simulink model "segway_completo"  (R2023b)
settings: Solver=ode45  StartTime=0.0  StopTime=8  MaxStep=1e-3  RelTol=1e-9  AbsTol=1e-11
values from neighbouring files (symbols this model uses):
  acople_rotor = p.e_acople    [INICIAR_SEGWAY.m]
  b_eje_mecanico = p.b_eje_mecanico    [INICIAR_SEGWAY.m]
  b_m_motor = motor.b_m    / motor.n_motores    [INICIAR_SEGWAY.m]
  b_phi = p.b_phi    [INICIAR_SEGWAY.m]
  b_x = p.b_x    [INICIAR_SEGWAY.m]
  beta_V_motor = motor.beta_V / motor.n_motores    [INICIAR_SEGWAY.m]
  compensar_delta_G = 1    [INICIAR_SEGWAY.m]
  giro_ref = 0    [INICIAR_SEGWAY.m]
  K = C.K    [INICIAR_SEGWAY.m]
  Kp_servo = 12    [INICIAR_SEGWAY.m]
  omega0 = 0    [INICIAR_SEGWAY.m]
  phi0 = deg2rad(5)    [INICIAR_SEGWAY.m]
  r = p.r    [INICIAR_SEGWAY.m]
  ruido_encoder_v = 0    [INICIAR_SEGWAY.m]
  ruido_encoder_x = 0    [INICIAR_SEGWAY.m]
  ruido_imu_angulo = 0    [INICIAR_SEGWAY.m]
  ruido_imu_giro = 0    [INICIAR_SEGWAY.m]
  sesgo_imu = 0    [INICIAR_SEGWAY.m]
  t_consigna = 2.0    (= 2)    [INICIAR_SEGWAY.m]
  t_patas = 4.0    (= 4)    [INICIAR_SEGWAY.m]
  tabla_a = zeros(size(tabla_theta))    [INICIAR_SEGWAY.m]
  tabla_delta_G = zeros(size(tabla_theta))    [INICIAR_SEGWAY.m]
  tabla_h = zeros(size(tabla_theta))    [INICIAR_SEGWAY.m]
  tabla_j = zeros(size(tabla_theta))    [INICIAR_SEGWAY.m]
  tabla_k = zeros(size(tabla_theta))    [INICIAR_SEGWAY.m]
  tabla_theta = deg2rad(grados_tabla(:))    [INICIAR_SEGWAY.m]
  tau_traccion = limite_de_traccion(p)    [INICIAR_SEGWAY.m]
  theta_pata_0 = deg2rad(postura_deg)    [INICIAR_SEGWAY.m]
  theta_pata_fin = deg2rad(theta_pata_fin)    [INICIAR_SEGWAY.m]
  theta_pata_max = (360 - min(fisicos.th))*pi/180    [INICIAR_SEGWAY.m]
  theta_pata_min = (360 - max(fisicos.th))*pi/180    [INICIAR_SEGWAY.m]
  Ts_sensores = 0.005    [INICIAR_SEGWAY.m]
  v0 = 0    [INICIAR_SEGWAY.m]
  V_bat = motor.V_bat    [INICIAR_SEGWAY.m]
  w_servo_max = deg2rad(300)    [INICIAR_SEGWAY.m]
  x0 = 0    [INICIAR_SEGWAY.m]
  x_destino = 0.30    (= 0.3)    [INICIAR_SEGWAY.m]
libraries: simulink x2
settings Model: Creator=calde  LastModifiedBy=calde

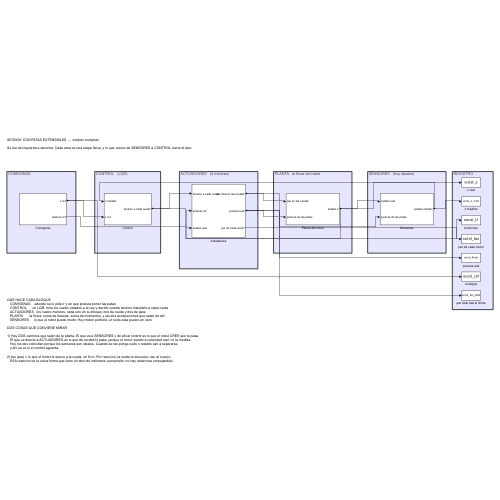
[thumbnail: Simulink's stored preview of the top-level diagram]
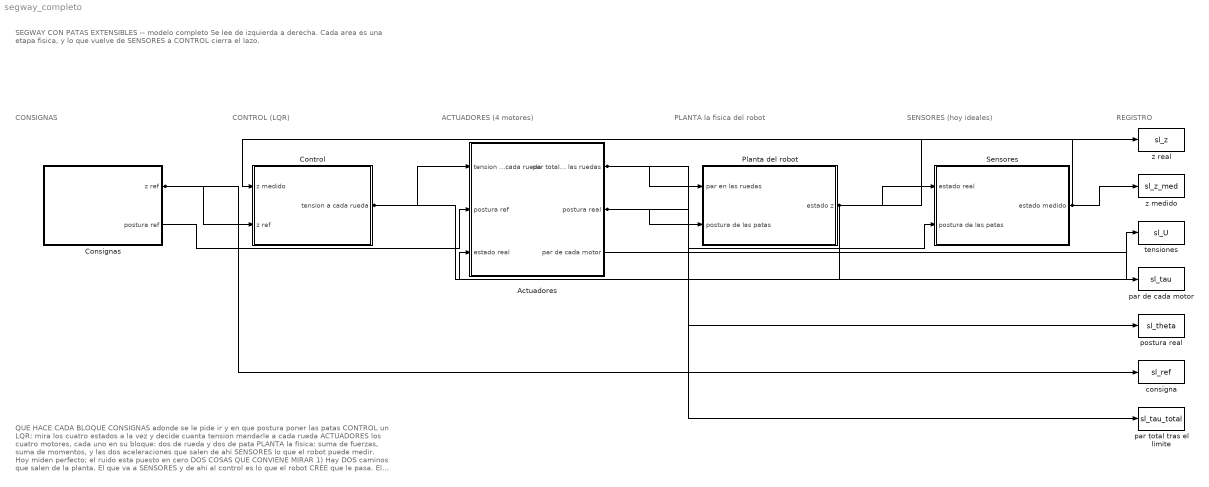
== system segway_completo ==
  note: CONSIGNAS
  note: CONTROL (LQR)
  note: ACTUADORES (4 motores)
  note: PLANTA la fisica del robot
  note: SENSORES (hoy ideales)
  note: REGISTRO
  note: SEGWAY CON PATAS EXTENSIBLES  --  modelo completo
      |
      | Se lee de izquierda a derecha. Cada area es una etapa fisica, y lo que vuelve de SENSORES a CONTROL cierra el lazo.
  note: QUE HACE CADA BLOQUE
      |    CONSIGNAS    adonde se le pide ir y en que postura poner las patas
      |    CONTROL      un LQR: mira los cuatro estados a la vez y decide cuanta tension mandarle a cada rueda
      |    ACTUADORES   los cuatro motores, cada uno en su bloque: dos de rueda y dos de pata
      |    PLANTA       la fisica: suma de fuerzas, suma de momentos, y las dos aceleraciones que salen de ahi
      |    SENSORES     lo que el robot puede medir. Hoy miden perfecto; el ruido esta puesto en cero
      |
      | DOS COSAS QUE CONVIENE MIRAR
      |
      | 1) Hay DOS caminos que salen de la planta. El que va a SENSORES y de ahi al control es lo que el robot CREE que le pasa.
      |    El que va directo a ACTUADORES es lo que de verdad le pasa, porque el motor siente la velocidad real, no la medida.
      |    Hoy los dos coinciden porque los sensores son ideales. Cuando se les ponga ruido o retardo van a separarse,
      |    y ahi se ve si el control aguanta.
      |
      | 2) tau (par) = lo que el motor le tuerce a la rueda, en N m. Por reaccion, la rueda le devuelve -tau al cuerpo.
      |    ESA reaccion es la unica forma que tiene el robot de inclinarse a proposito: no hay nada mas empujandolo.
  Actuadores : Subsystem
  Consignas : Subsystem
  Control : Subsystem
  Planta del robot : Subsystem
  Sensores : Subsystem
  consigna : ToWorkspace  VariableName=sl_ref  SaveFormat=Structure With Time  SampleTime=-1
  par de cada motor : ToWorkspace  VariableName=sl_tau  SaveFormat=Structure With Time  SampleTime=-1
  par total tras el limite : ToWorkspace  VariableName=sl_tau_total  SaveFormat=Structure With Time  SampleTime=-1
  postura real : ToWorkspace  VariableName=sl_theta  SaveFormat=Structure With Time  SampleTime=-1
  tensiones : ToWorkspace  VariableName=sl_U  SaveFormat=Structure With Time  SampleTime=-1
  z medido : ToWorkspace  VariableName=sl_z_med  SaveFormat=Structure With Time  SampleTime=-1
  z real : ToWorkspace  VariableName=sl_z  SaveFormat=Structure With Time  SampleTime=-1
  wires:
  Consignas/1(z ref) -> Control/2(z ref), consigna/1
  Consignas/2(postura ref) -> Actuadores/2(postura ref)
  Sensores/1(estado medido) -> Control/1(z medido), z medido/1
  Control/1(tension a cada rueda) -> Actuadores/1(tension a cada rueda), tensiones/1
  Planta del robot/1(estado z) -> Actuadores/3(estado real), Sensores/1(estado real), z real/1
  Actuadores/1(par total en las ruedas) -> Planta del robot/1(par en las ruedas), par total tras el limite/1
  Actuadores/2(postura real) -> Planta del robot/2(postura de las patas), Sensores/2(postura de las patas), postura real/1
  Actuadores/3(par de cada motor) -> par de cada motor/1

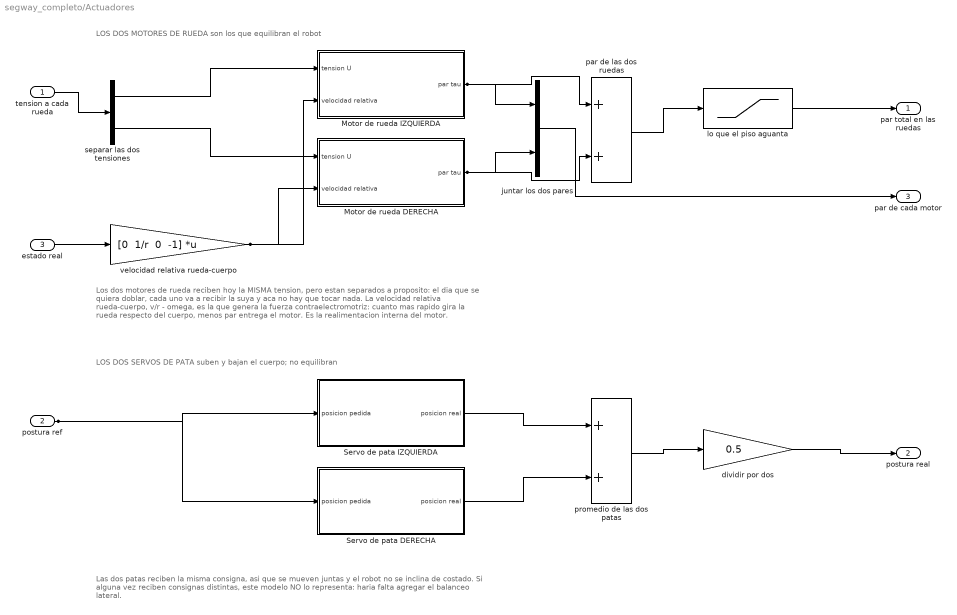
== system segway_completo/Actuadores ==
  note: LOS DOS MOTORES DE RUEDA son los que equilibran el robot
  note: LOS DOS SERVOS DE PATA suben y bajan el cuerpo; no equilibran
  note: Los dos motores de rueda reciben hoy la MISMA tension, pero estan separados a proposito: el dia que se
      | quiera doblar, cada uno va a recibir la suya y aca no hay que tocar nada.
      |
      | La velocidad relativa rueda-cuerpo, v/r - omega, es la que genera la fuerza contraelectromotriz: cuanto mas
      | rapido gira la rueda respecto del cuerpo, menos par entrega el motor. Es la realimentacion interna del motor.
  note: Las dos patas reciben la misma consigna, asi que se mueven juntas y el robot no se inclina de costado.
      | Si alguna vez reciben consignas distintas, este modelo NO lo representa: haria falta agregar el balanceo lateral.
  tension a cada rueda : Inport
  postura ref : Inport  Port=2
  estado real : Inport  Port=3
  Motor de rueda DERECHA : Subsystem
  Motor de rueda IZQUIERDA : Subsystem
  Servo de pata DERECHA : Subsystem
  Servo de pata IZQUIERDA : Subsystem
  dividir por dos : Gain  Gain=0.5
  juntar los dos pares : Mux  Inputs=2
  lo que el piso aguanta : Saturate  UpperLimit=tau_traccion  LowerLimit=-tau_traccion
  par de las dos ruedas : Sum
  promedio de las dos patas : Sum
  separar las dos tensiones : Demux  Outputs=2
  velocidad relativa rueda-cuerpo : Gain  Gain="[0  1/r  0  -1]"  Multiplication=Matrix(K*u)
  par total en las ruedas : Outport
  postura real : Outport  Port=2
  par de cada motor : Outport  Port=3
  wires:
  tension a cada rueda/1 -> separar las dos tensiones/1
  estado real/1 -> velocidad relativa rueda-cuerpo/1
  separar las dos tensiones/1 -> Motor de rueda IZQUIERDA/1(tension U)
  separar las dos tensiones/2 -> Motor de rueda DERECHA/1(tension U)
  velocidad relativa rueda-cuerpo/1 -> Motor de rueda IZQUIERDA/2(velocidad relativa), Motor de rueda DERECHA/2(velocidad relativa)
  Motor de rueda IZQUIERDA/1(par tau) -> par de las dos ruedas/1, juntar los dos pares/1
  Motor de rueda DERECHA/1(par tau) -> par de las dos ruedas/2, juntar los dos pares/2
  juntar los dos pares/1 -> par de cada motor/1
  par de las dos ruedas/1 -> lo que el piso aguanta/1
  lo que el piso aguanta/1 -> par total en las ruedas/1
  postura ref/1 -> Servo de pata IZQUIERDA/1(posicion pedida), Servo de pata DERECHA/1(posicion pedida)
  Servo de pata IZQUIERDA/1(posicion real) -> promedio de las dos patas/1
  Servo de pata DERECHA/1(posicion real) -> promedio de las dos patas/2
  promedio de las dos patas/1 -> dividir por dos/1
  dividir por dos/1 -> postura real/1

== system segway_completo/Consignas ==
  note: EQUILIBRIO Y POSICION: z_ref = [x deseado ; 0 ; 0 ; 0]
  note: PATAS: angulo pedido al servo, en radianes (10 grados = plegada, 40 = estirada)
  note: Por defecto la postura es constante, asi que el robot se comporta como el modelo verificado.
      | Si se le pone un escalon (theta_pata_fin distinto de theta_pata_0) las patas se mueven y
      | cambian la altura del cuerpo: ver el capitulo 9 del PDF del modelo.
  adonde ir : Step  Time=t_consigna  After=x_destino  SampleTime=0
  armar z ref : Mux  Inputs=2
  postura de las patas : Step  Time=t_patas  Before=theta_pata_0  After=theta_pata_fin  SampleTime=0
  "velocidad, angulo y giro pedidos" : Constant  Value=[0; 0; 0]
  z ref : Outport
  postura ref : Outport  Port=2
  wires:
  adonde ir/1 -> armar z ref/1
  "velocidad, angulo y giro pedidos"/1 -> armar z ref/2
  armar z ref/1 -> z ref/1
  postura de las patas/1 -> postura ref/1

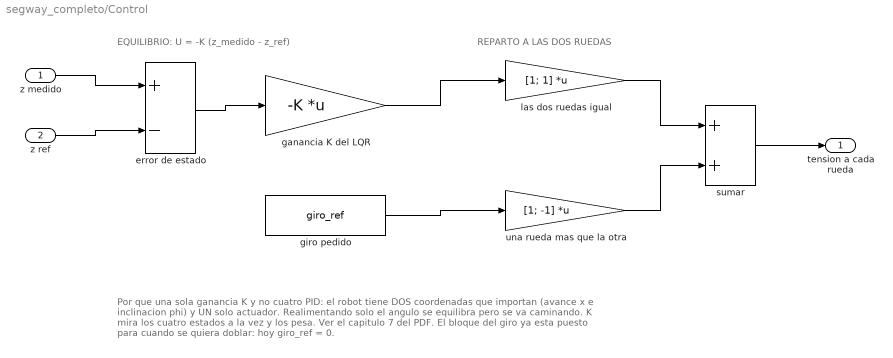
== system segway_completo/Control ==
  note: EQUILIBRIO: U = -K (z_medido - z_ref)
  note: REPARTO A LAS DOS RUEDAS
  note: Por que una sola ganancia K y no cuatro PID: el robot tiene DOS coordenadas que importan
      | (avance x e inclinacion phi) y UN solo actuador. Realimentando solo el angulo se equilibra
      | pero se va caminando. K mira los cuatro estados a la vez y los pesa. Ver el capitulo 7 del PDF.
      |
      | El bloque del giro ya esta puesto para cuando se quiera doblar: hoy giro_ref = 0.
  z medido : Inport
  z ref : Inport  Port=2
  error de estado : Sum  Inputs=+-
  ganancia K del LQR : Gain  Gain=-K  Multiplication=Matrix(K*u)
  giro pedido : Constant  Value=giro_ref
  las dos ruedas igual : Gain  Gain=[1; 1]  Multiplication=Matrix(K*u)
  sumar : Sum
  una rueda mas que la otra : Gain  Gain=[1; -1]  Multiplication=Matrix(K*u)
  tension a cada rueda : Outport
  wires:
  z medido/1 -> error de estado/1
  z ref/1 -> error de estado/2
  error de estado/1 -> ganancia K del LQR/1
  ganancia K del LQR/1 -> las dos ruedas igual/1
  giro pedido/1 -> una rueda mas que la otra/1
  las dos ruedas igual/1 -> sumar/1
  una rueda mas que la otra/1 -> sumar/2
  sumar/1 -> tension a cada rueda/1

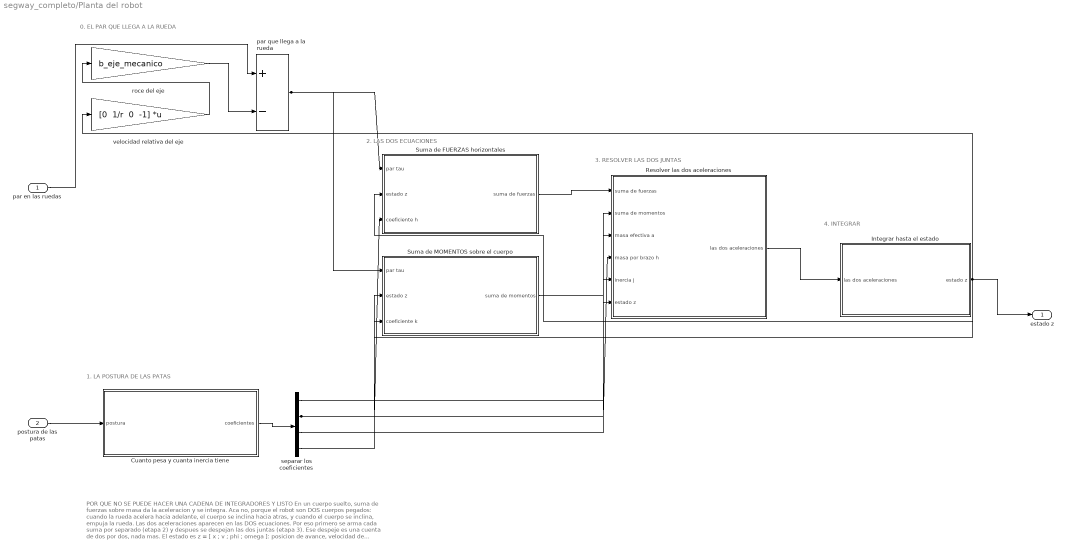
== system segway_completo/Planta del robot ==
  note: 1. LA POSTURA DE LAS PATAS
  note: 0. EL PAR QUE LLEGA A LA RUEDA
  note: 2. LAS DOS ECUACIONES
  note: 3. RESOLVER LAS DOS JUNTAS
  note: 4. INTEGRAR
  note: POR QUE NO SE PUEDE HACER UNA CADENA DE INTEGRADORES Y LISTO
      |
      | En un cuerpo suelto, suma de fuerzas sobre masa da la aceleracion y se integra. Aca no, porque el robot son DOS cuerpos
      | pegados: cuando la rueda acelera hacia adelante, el cuerpo se inclina hacia atras, y cuando el cuerpo se inclina, empuja
      | la rueda. Las dos aceleraciones aparecen en las DOS ecuaciones. Por eso primero se arma cada suma por separado (etapa 2)
      | y despues se despejan las dos juntas (etapa 3). Ese despeje es una cuenta de dos por dos, nada mas.
      |
      | El estado es  z = [ x ; v ; phi ; omega ]:  posicion de avance, velocidad de avance, inclinacion y velocidad de inclinacion.
  par en las ruedas : Inport
  postura de las patas : Inport  Port=2
  Cuanto pesa y cuanta inercia tiene : Subsystem
  Integrar hasta el estado : Subsystem
  Resolver las dos aceleraciones : Subsystem
  Suma de FUERZAS horizontales : Subsystem
  Suma de MOMENTOS sobre el cuerpo : Subsystem
  par que llega a la rueda : Sum  Inputs=+-
  roce del eje : Gain  Gain=b_eje_mecanico
  separar los coeficientes : Demux
  velocidad relativa del eje : Gain  Gain="[0  1/r  0  -1]"  Multiplication=Matrix(K*u)
  estado z : Outport
  wires:
  postura de las patas/1 -> Cuanto pesa y cuanta inercia tiene/1(postura)
  Cuanto pesa y cuanta inercia tiene/1(coeficientes) -> separar los coeficientes/1
  Integrar hasta el estado/1(estado z) -> velocidad relativa del eje/1, Suma de FUERZAS horizontales/2(estado z), Suma de MOMENTOS sobre el cuerpo/2(estado z), Resolver las dos aceleraciones/6(estado z), estado z/1
  velocidad relativa del eje/1 -> roce del eje/1
  par en las ruedas/1 -> par que llega a la rueda/1
  roce del eje/1 -> par que llega a la rueda/2
  par que llega a la rueda/1 -> Suma de FUERZAS horizontales/1(par tau), Suma de MOMENTOS sobre el cuerpo/1(par tau)
  separar los coeficientes/2 -> Suma de FUERZAS horizontales/3(coeficiente h), Resolver las dos aceleraciones/4(masa por brazo h)
  separar los coeficientes/4 -> Suma de MOMENTOS sobre el cuerpo/3(coeficiente k)
  Suma de FUERZAS horizontales/1(suma de fuerzas) -> Resolver las dos aceleraciones/1(suma de fuerzas)
  Suma de MOMENTOS sobre el cuerpo/1(suma de momentos) -> Resolver las dos aceleraciones/2(suma de momentos)
  separar los coeficientes/1 -> Resolver las dos aceleraciones/3(masa efectiva a)
  separar los coeficientes/3 -> Resolver las dos aceleraciones/5(inercia j)
  Resolver las dos aceleraciones/1(las dos aceleraciones) -> Integrar hasta el estado/1(las dos aceleraciones)

== system segway_completo/Sensores ==
  note: ENCODERS: x y v
  note: IMU: phi y omega
  note: HOY LOS SENSORES SON IDEALES: miden exactamente lo que pasa y el ruido esta en cero. Por eso la senal que
      | entra al control es identica a la real, y el resultado coincide con el modelo matematico.
      |
      | Los lugares donde meter la realidad ya estan puestos:
      |   - ruido: las variables ruido_* valen cero; poniendoles un numero aparece el ruido de medicion
      |   - sesgo de la IMU: sesgo_imu, en radianes
      |   - compensacion de la postura: compensar_delta_G vale 1; poniendolo en 0 se ve el error de no corregirla
      |
      | Lo que TODAVIA no esta y hay que agregar antes de pasar a firmware: periodo de muestreo, retardo de calculo
      | y cuantizacion del encoder. Con esos tres el LQR hubo que repesarlo (capitulo 7 del PDF).
  estado real : Inport
  postura de las patas : Inport  Port=2
  Encoders de las ruedas : Subsystem
  IMU MPU-6050 : Subsystem
  armar el estado medido : Mux  Inputs=2
  estado medido : Outport
  wires:
  estado real/1 -> Encoders de las ruedas/1(estado real), IMU MPU-6050/1(estado real)
  postura de las patas/1 -> IMU MPU-6050/2(postura de las patas)
  Encoders de las ruedas/1(x y v medidos) -> armar el estado medido/1
  IMU MPU-6050/1(phi y omega medidos) -> armar el estado medido/2
  armar el estado medido/1 -> estado medido/1

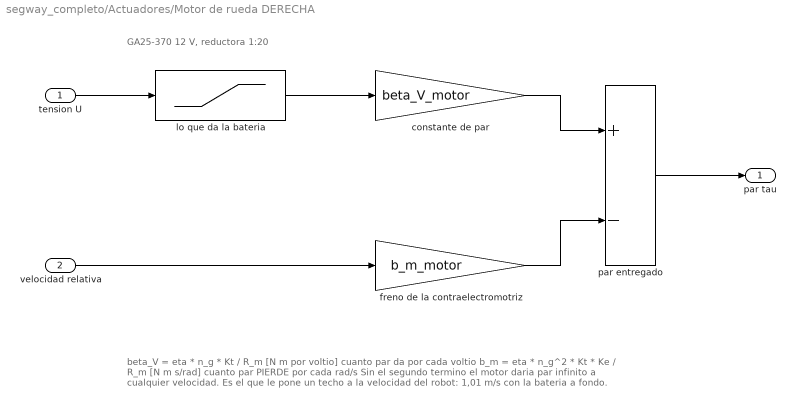
== system segway_completo/Actuadores/Motor de rueda DERECHA ==
  note: GA25-370 12 V, reductora 1:20
  note: beta_V = eta * n_g * Kt / R_m   [N m por voltio]        cuanto par da por cada voltio
      | b_m    = eta * n_g^2 * Kt * Ke / R_m   [N m s/rad]      cuanto par PIERDE por cada rad/s
      |
      | Sin el segundo termino el motor daria par infinito a cualquier velocidad. Es el que le pone
      | un techo a la velocidad del robot: 1,01 m/s con la bateria a fondo.
  tension U : Inport
  velocidad relativa : Inport  Port=2
  constante de par : Gain  Gain=beta_V_motor
  freno de la contraelectromotriz : Gain  Gain=b_m_motor
  lo que da la bateria : Saturate  UpperLimit=V_bat  LowerLimit=-V_bat
  par entregado : Sum  Inputs=+-
  par tau : Outport
  wires:
  tension U/1 -> lo que da la bateria/1
  lo que da la bateria/1 -> constante de par/1
  velocidad relativa/1 -> freno de la contraelectromotriz/1
  constante de par/1 -> par entregado/1
  freno de la contraelectromotriz/1 -> par entregado/2
  par entregado/1 -> par tau/1

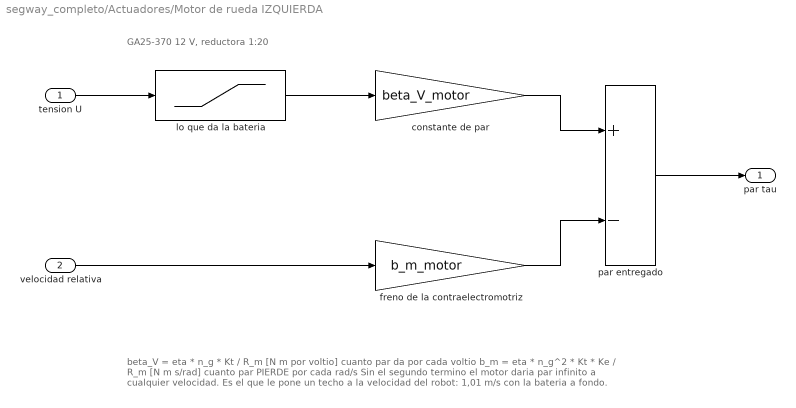
== system segway_completo/Actuadores/Motor de rueda IZQUIERDA ==
  note: GA25-370 12 V, reductora 1:20
  note: beta_V = eta * n_g * Kt / R_m   [N m por voltio]        cuanto par da por cada voltio
      | b_m    = eta * n_g^2 * Kt * Ke / R_m   [N m s/rad]      cuanto par PIERDE por cada rad/s
      |
      | Sin el segundo termino el motor daria par infinito a cualquier velocidad. Es el que le pone
      | un techo a la velocidad del robot: 1,01 m/s con la bateria a fondo.
  tension U : Inport
  velocidad relativa : Inport  Port=2
  constante de par : Gain  Gain=beta_V_motor
  freno de la contraelectromotriz : Gain  Gain=b_m_motor
  lo que da la bateria : Saturate  UpperLimit=V_bat  LowerLimit=-V_bat
  par entregado : Sum  Inputs=+-
  par tau : Outport
  wires:
  tension U/1 -> lo que da la bateria/1
  lo que da la bateria/1 -> constante de par/1
  velocidad relativa/1 -> freno de la contraelectromotriz/1
  constante de par/1 -> par entregado/1
  freno de la contraelectromotriz/1 -> par entregado/2
  par entregado/1 -> par tau/1

== system segway_completo/Actuadores/Servo de pata DERECHA ==
  note: DS3240 40 kg cm: lazo de posicion
  note: Un servo de posicion ya trae su propio control adentro: por eso aca no hay que disenarle nada,
      | solo decirle a que angulo ir. El lazo que se ve es el que el servo tiene de fabrica.
      |
      | Los topes del integrador son los topes MECANICOS de la pata: 10 grados plegada, 40 estirada.
      | Que esten en el integrador y no en una saturacion aparte evita que el angulo se pase y despues vuelva.
  posicion pedida : Inport
  angulo de la pata : Integrator  InitialCondition=theta_pata_0  LimitOutput=on  UpperSaturationLimit=theta_pata_max  LowerSaturationLimit=theta_pata_min
  error de posicion : Sum  Inputs=+-
  ganancia del servo : Gain  Gain=Kp_servo
  velocidad maxima : Saturate  UpperLimit=w_servo_max  LowerLimit=-w_servo_max
  posicion real : Outport
  wires:
  posicion pedida/1 -> error de posicion/1
  ganancia del servo/1 -> velocidad maxima/1
  error de posicion/1 -> ganancia del servo/1
  velocidad maxima/1 -> angulo de la pata/1
  angulo de la pata/1 -> posicion real/1, error de posicion/2

== system segway_completo/Actuadores/Servo de pata IZQUIERDA ==
  note: DS3240 40 kg cm: lazo de posicion
  note: Un servo de posicion ya trae su propio control adentro: por eso aca no hay que disenarle nada,
      | solo decirle a que angulo ir. El lazo que se ve es el que el servo tiene de fabrica.
      |
      | Los topes del integrador son los topes MECANICOS de la pata: 10 grados plegada, 40 estirada.
      | Que esten en el integrador y no en una saturacion aparte evita que el angulo se pase y despues vuelva.
  posicion pedida : Inport
  angulo de la pata : Integrator  InitialCondition=theta_pata_0  LimitOutput=on  UpperSaturationLimit=theta_pata_max  LowerSaturationLimit=theta_pata_min
  error de posicion : Sum  Inputs=+-
  ganancia del servo : Gain  Gain=Kp_servo
  velocidad maxima : Saturate  UpperLimit=w_servo_max  LowerLimit=-w_servo_max
  posicion real : Outport
  wires:
  posicion pedida/1 -> error de posicion/1
  ganancia del servo/1 -> velocidad maxima/1
  error de posicion/1 -> ganancia del servo/1
  velocidad maxima/1 -> angulo de la pata/1
  angulo de la pata/1 -> posicion real/1, error de posicion/2

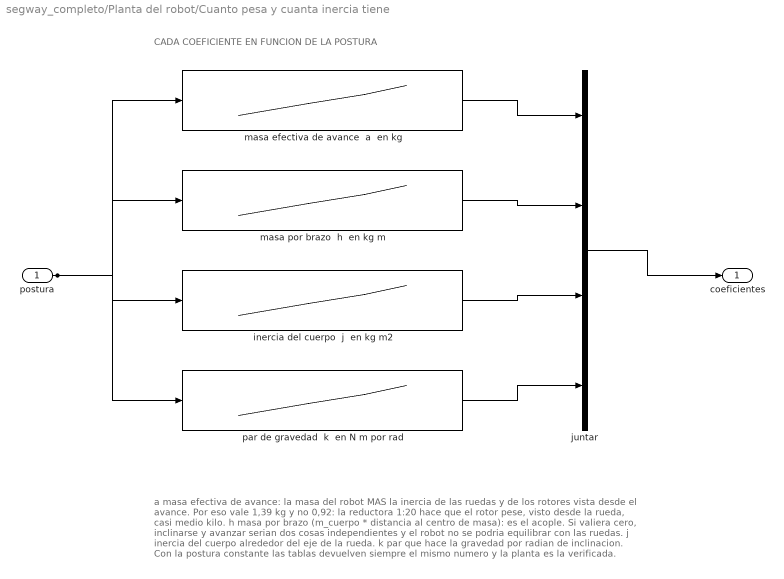
== system segway_completo/Planta del robot/Cuanto pesa y cuanta inercia tiene ==
  note: CADA COEFICIENTE EN FUNCION DE LA POSTURA
  note: a  masa efectiva de avance: la masa del robot MAS la inercia de las ruedas y de los rotores vista desde el avance.
      |    Por eso vale 1,39 kg y no 0,92: la reductora 1:20 hace que el rotor pese, visto desde la rueda, casi medio kilo.
      |
      | h  masa por brazo (m_cuerpo * distancia al centro de masa): es el acople. Si valiera cero, inclinarse y avanzar
      |    serian dos cosas independientes y el robot no se podria equilibrar con las ruedas.
      |
      | j  inercia del cuerpo alrededor del eje de la rueda.      k  par que hace la gravedad por radian de inclinacion.
      |
      | Con la postura constante las tablas devuelven siempre el mismo numero y la planta es la verificada.
  postura : Inport
  inercia del cuerpo  j  en kg m2 : Lookup_n-D  NumberOfTableDimensions=1  BreakpointsForDimension1=tabla_theta  Table=tabla_j  InternalRulePriority=Speed  RndMeth=Simplest
  juntar : Mux
  masa efectiva de avance  a  en kg : Lookup_n-D  NumberOfTableDimensions=1  BreakpointsForDimension1=tabla_theta  Table=tabla_a  InternalRulePriority=Speed  RndMeth=Simplest
  masa por brazo  h  en kg m : Lookup_n-D  NumberOfTableDimensions=1  BreakpointsForDimension1=tabla_theta  Table=tabla_h  InternalRulePriority=Speed  RndMeth=Simplest
  par de gravedad  k  en N m por rad : Lookup_n-D  NumberOfTableDimensions=1  BreakpointsForDimension1=tabla_theta  Table=tabla_k  InternalRulePriority=Speed  RndMeth=Simplest
  coeficientes : Outport
  wires:
  postura/1 -> masa efectiva de avance  a  en kg/1, masa por brazo  h  en kg m/1, inercia del cuerpo  j  en kg m2/1, par de gravedad  k  en N m por rad/1
  masa efectiva de avance  a  en kg/1 -> juntar/1
  masa por brazo  h  en kg m/1 -> juntar/2
  inercia del cuerpo  j  en kg m2/1 -> juntar/3
  par de gravedad  k  en N m por rad/1 -> juntar/4
  juntar/1 -> coeficientes/1

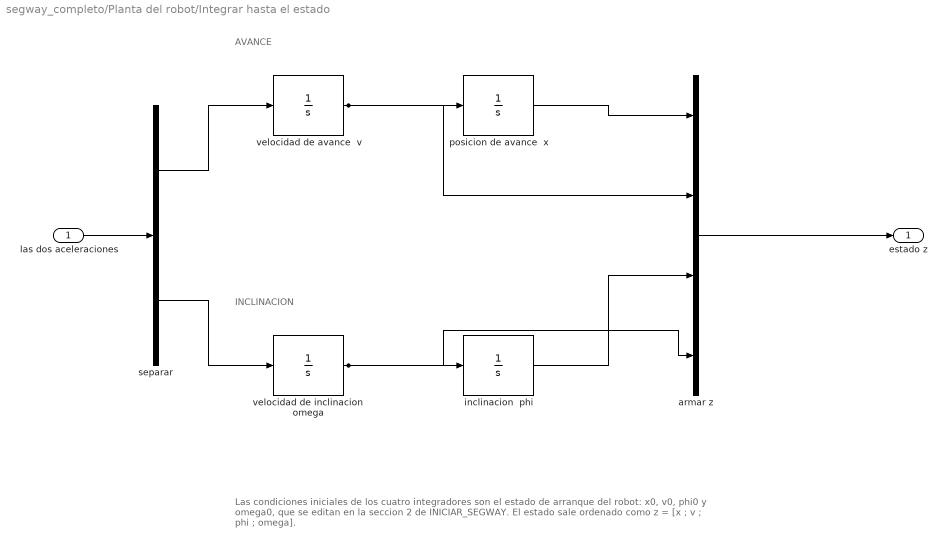
== system segway_completo/Planta del robot/Integrar hasta el estado ==
  note: AVANCE
  note: INCLINACION
  note: Las condiciones iniciales de los cuatro integradores son el estado de arranque del robot:
      | x0, v0, phi0 y omega0, que se editan en la seccion 2 de INICIAR_SEGWAY.
      | El estado sale ordenado como z = [x ; v ; phi ; omega].
  las dos aceleraciones : Inport
  armar z : Mux
  inclinacion  phi : Integrator  InitialCondition=phi0
  posicion de avance  x : Integrator  InitialCondition=x0
  separar : Demux  Outputs=2
  velocidad de avance  v : Integrator  InitialCondition=v0
  velocidad de inclinacion  omega : Integrator  InitialCondition=omega0
  estado z : Outport
  wires:
  las dos aceleraciones/1 -> separar/1
  separar/1 -> velocidad de avance  v/1
  velocidad de avance  v/1 -> posicion de avance  x/1, armar z/2
  separar/2 -> velocidad de inclinacion  omega/1
  velocidad de inclinacion  omega/1 -> inclinacion  phi/1, armar z/4
  posicion de avance  x/1 -> armar z/1
  inclinacion  phi/1 -> armar z/3
  armar z/1 -> estado z/1

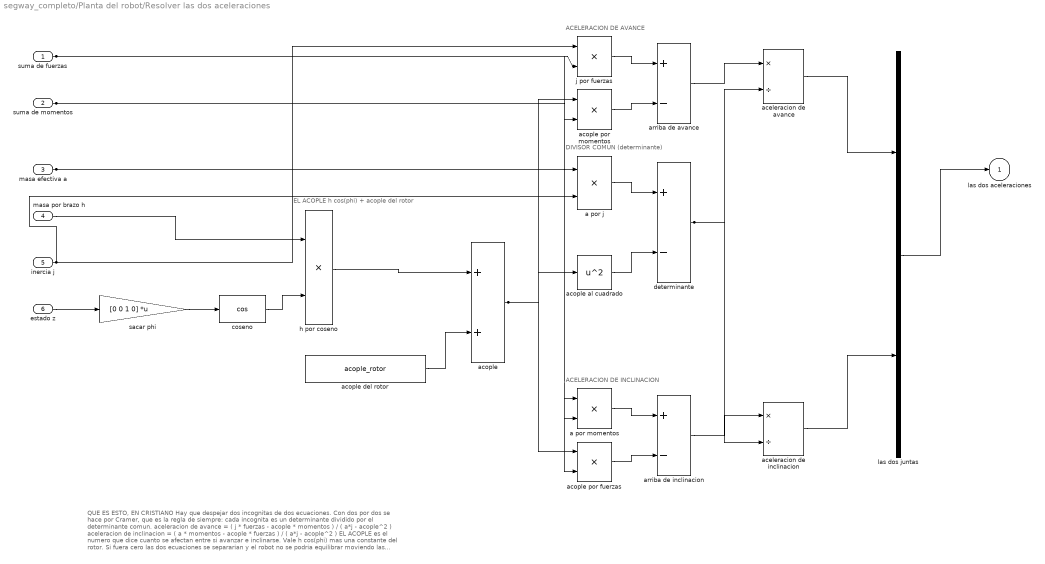
== system segway_completo/Planta del robot/Resolver las dos aceleraciones ==
  note: EL ACOPLE h cos(phi) + acople del rotor
  note: ACELERACION DE AVANCE
  note: DIVISOR COMUN (determinante)
  note: ACELERACION DE INCLINACION
  note: QUE ES ESTO, EN CRISTIANO
      |
      | Hay que despejar dos incognitas de dos ecuaciones. Con dos por dos se hace por Cramer, que es la regla
      | de siempre: cada incognita es un determinante dividido por el determinante comun.
      |
      |   aceleracion de avance      = ( j * fuerzas  -  acople * momentos ) / ( a*j - acople^2 )
      |   aceleracion de inclinacion = ( a * momentos -  acople * fuerzas  ) / ( a*j - acople^2 )
      |
      | EL ACOPLE es el numero que dice cuanto se afectan entre si avanzar e inclinarse. Vale h cos(phi) mas una
      | constante del rotor. Si fuera cero las dos ecuaciones se separarian y el robot no se podria equilibrar
      | moviendo las ruedas, porque empujar la rueda no inclinaria el cuerpo.
  suma de fuerzas : Inport
  suma de momentos : Inport  Port=2
  masa efectiva a : Inport  Port=3
  masa por brazo h : Inport  Port=4
  inercia j : Inport  Port=5
  estado z : Inport  Port=6
  a por j : Product
  a por momentos : Product
  aceleracion de avance : Product  Inputs=*/
  aceleracion de inclinacion : Product  Inputs=*/
  acople : Sum
  acople al cuadrado : Math  Operator=square
  acople del rotor : Constant  Value=acople_rotor
  acople por fuerzas : Product
  acople por momentos : Product
  arriba de avance : Sum  Inputs=+-
  arriba de inclinacion : Sum  Inputs=+-
  coseno : Trigonometry  Operator=cos
  determinante : Sum  Inputs=+-
  h por coseno : Product
  j por fuerzas : Product
  las dos juntas : Mux  Inputs=2
  sacar phi : Gain  Gain=[0 0 1 0]  Multiplication=Matrix(K*u)
  las dos aceleraciones : Outport
  wires:
  estado z/1 -> sacar phi/1
  sacar phi/1 -> coseno/1
  masa por brazo h/1 -> h por coseno/1
  coseno/1 -> h por coseno/2
  h por coseno/1 -> acople/1
  acople del rotor/1 -> acople/2
  masa efectiva a/1 -> a por j/1, a por momentos/1
  inercia j/1 -> a por j/2, j por fuerzas/1
  acople/1 -> acople al cuadrado/1, acople por momentos/1, acople por fuerzas/1
  a por j/1 -> determinante/1
  acople al cuadrado/1 -> determinante/2
  suma de fuerzas/1 -> j por fuerzas/2, acople por fuerzas/2
  suma de momentos/1 -> acople por momentos/2, a por momentos/2
  j por fuerzas/1 -> arriba de avance/1
  acople por momentos/1 -> arriba de avance/2
  a por momentos/1 -> arriba de inclinacion/1
  acople por fuerzas/1 -> arriba de inclinacion/2
  arriba de avance/1 -> aceleracion de avance/1
  determinante/1 -> aceleracion de avance/2, aceleracion de inclinacion/2
  arriba de inclinacion/1 -> aceleracion de inclinacion/1
  aceleracion de avance/1 -> las dos juntas/1
  aceleracion de inclinacion/1 -> las dos juntas/2
  las dos juntas/1 -> las dos aceleraciones/1

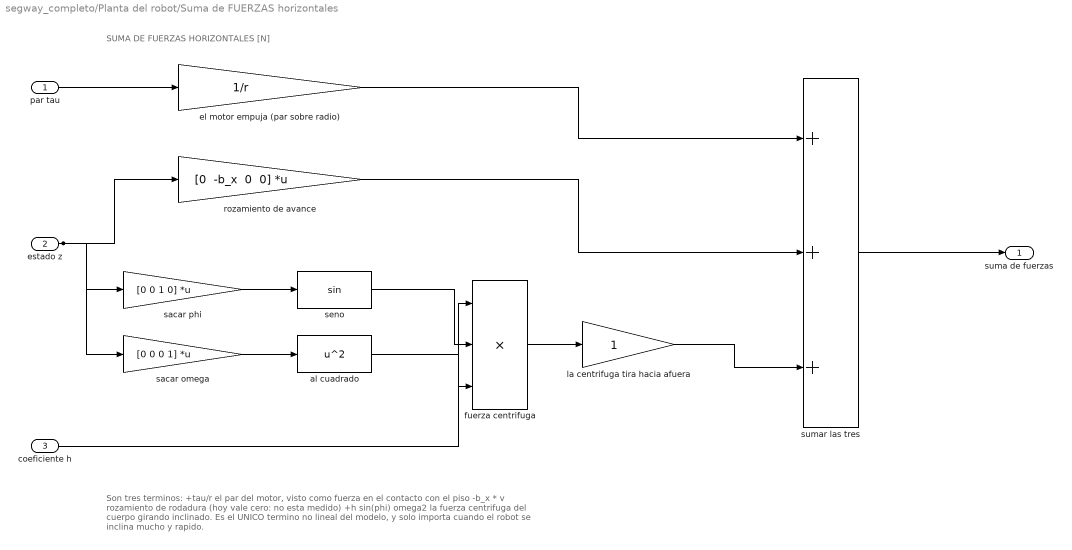
== system segway_completo/Planta del robot/Suma de FUERZAS horizontales ==
  note: SUMA DE FUERZAS HORIZONTALES [N]
  note: Son tres terminos:
      |
      |   +tau/r             el par del motor, visto como fuerza en el contacto con el piso
      |   -b_x * v           rozamiento de rodadura (hoy vale cero: no esta medido)
      |   +h sin(phi) omega2 la fuerza centrifuga del cuerpo girando inclinado. Es el UNICO termino no lineal
      |                      del modelo, y solo importa cuando el robot se inclina mucho y rapido.
  par tau : Inport
  estado z : Inport  Port=2
  coeficiente h : Inport  Port=3
  al cuadrado : Math  Operator=square
  el motor empuja (par sobre radio) : Gain  Gain=1/r
  fuerza centrifuga : Product  Inputs=3
  la centrifuga tira hacia afuera : Gain
  rozamiento de avance : Gain  Gain="[0  -b_x  0  0]"  Multiplication=Matrix(K*u)
  sacar omega : Gain  Gain=[0 0 0 1]  Multiplication=Matrix(K*u)
  sacar phi : Gain  Gain=[0 0 1 0]  Multiplication=Matrix(K*u)
  seno : Trigonometry
  sumar las tres : Sum  Inputs=+++
  suma de fuerzas : Outport
  wires:
  par tau/1 -> el motor empuja (par sobre radio)/1
  estado z/1 -> rozamiento de avance/1, sacar phi/1, sacar omega/1
  sacar phi/1 -> seno/1
  sacar omega/1 -> al cuadrado/1
  coeficiente h/1 -> fuerza centrifuga/1
  seno/1 -> fuerza centrifuga/2
  al cuadrado/1 -> fuerza centrifuga/3
  fuerza centrifuga/1 -> la centrifuga tira hacia afuera/1
  el motor empuja (par sobre radio)/1 -> sumar las tres/1
  rozamiento de avance/1 -> sumar las tres/2
  la centrifuga tira hacia afuera/1 -> sumar las tres/3
  sumar las tres/1 -> suma de fuerzas/1

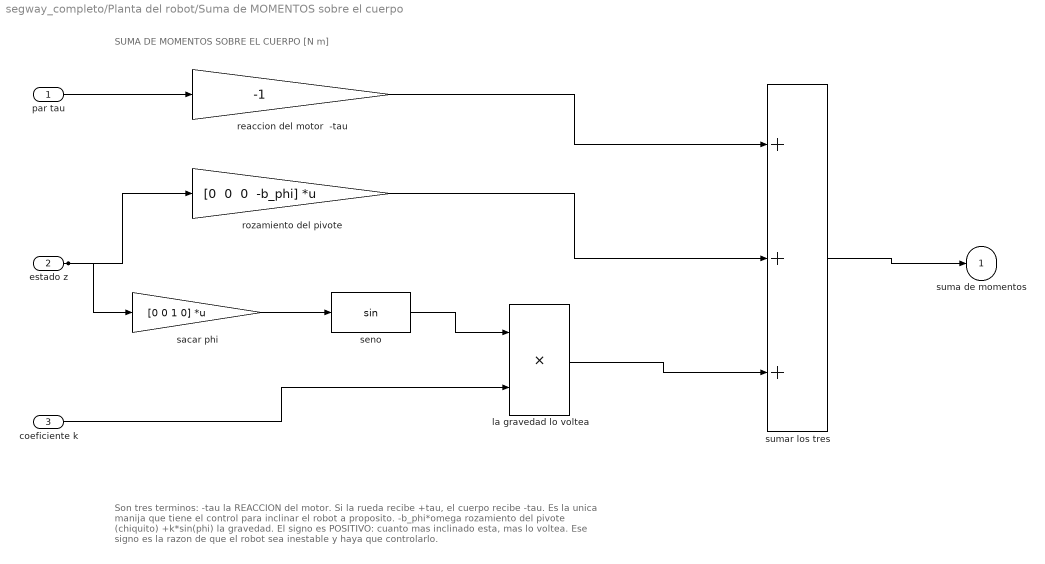
== system segway_completo/Planta del robot/Suma de MOMENTOS sobre el cuerpo ==
  note: SUMA DE MOMENTOS SOBRE EL CUERPO [N m]
  note: Son tres terminos:
      |
      |   -tau          la REACCION del motor. Si la rueda recibe +tau, el cuerpo recibe -tau. Es la unica
      |                 manija que tiene el control para inclinar el robot a proposito.
      |   -b_phi*omega  rozamiento del pivote (chiquito)
      |   +k*sin(phi)   la gravedad. El signo es POSITIVO: cuanto mas inclinado esta, mas lo voltea.
      |                 Ese signo es la razon de que el robot sea inestable y haya que controlarlo.
  par tau : Inport
  estado z : Inport  Port=2
  coeficiente k : Inport  Port=3
  la gravedad lo voltea : Product
  reaccion del motor  -tau : Gain  Gain=-1
  rozamiento del pivote : Gain  Gain="[0  0  0  -b_phi]"  Multiplication=Matrix(K*u)
  sacar phi : Gain  Gain=[0 0 1 0]  Multiplication=Matrix(K*u)
  seno : Trigonometry
  sumar los tres : Sum  Inputs=+++
  suma de momentos : Outport
  wires:
  par tau/1 -> reaccion del motor  -tau/1
  estado z/1 -> rozamiento del pivote/1, sacar phi/1
  sacar phi/1 -> seno/1
  seno/1 -> la gravedad lo voltea/1
  coeficiente k/1 -> la gravedad lo voltea/2
  reaccion del motor  -tau/1 -> sumar los tres/1
  rozamiento del pivote/1 -> sumar los tres/2
  la gravedad lo voltea/1 -> sumar los tres/3
  sumar los tres/1 -> suma de momentos/1

== system segway_completo/Sensores/Encoders de las ruedas ==
  note: ENCODER DE CUADRATURA
  note: RUIDO hoy en cero
  note: El encoder cuenta pulsos del eje del motor. Con la reductora 1:20 y la rueda de 33 mm, cada cuenta
      | son 0,29 mm de avance: de sobra para la posicion.
      |
      | El problema es la VELOCIDAD: a 0,1 m/s entran solo 2 cuentas por cada muestra de 5 ms. Por eso el
      | diseno del LQR ya tiene en cuenta un filtro de 20 Hz sobre la velocidad.
  estado real : Inport
  medicion : Sum
  ruido del encoder : simulink/Sources/Band-Limited White Noise  Cov="[ruido_encoder_x  ruido_encoder_v]"  Ts=Ts_sensores  seed=[41 43]
  sacar x y v de verdad : Gain  Gain=[1 0 0 0; 0 1 0 0]  Multiplication=Matrix(K*u)
  x y v medidos : Outport
  wires:
  estado real/1 -> sacar x y v de verdad/1
  sacar x y v de verdad/1 -> medicion/1
  ruido del encoder/1 -> medicion/2
  medicion/1 -> x y v medidos/1

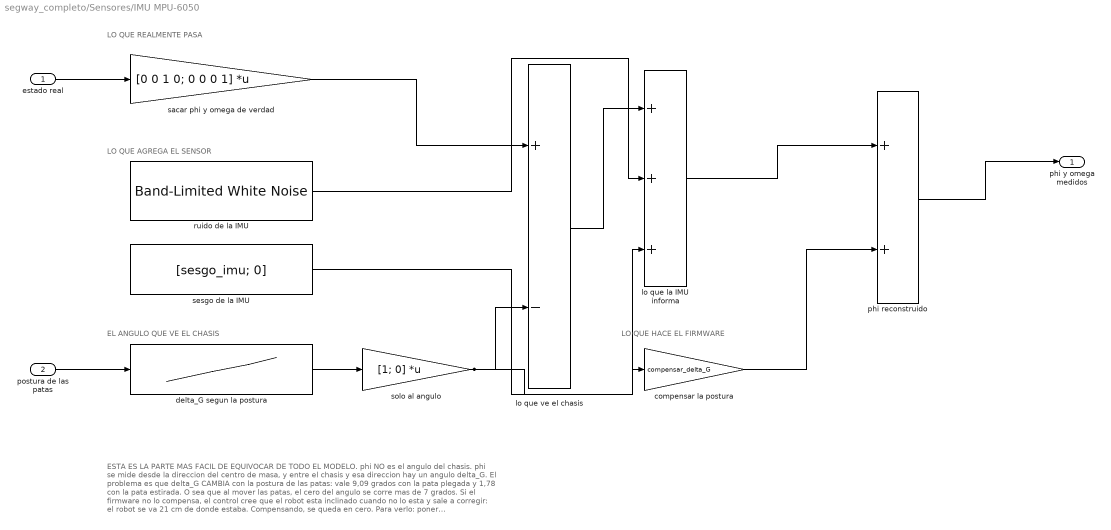
== system segway_completo/Sensores/IMU MPU-6050 ==
  note: LO QUE REALMENTE PASA
  note: LO QUE AGREGA EL SENSOR
  note: EL ANGULO QUE VE EL CHASIS
  note: LO QUE HACE EL FIRMWARE
  note: ESTA ES LA PARTE MAS FACIL DE EQUIVOCAR DE TODO EL MODELO.
      |
      | phi NO es el angulo del chasis. phi se mide desde la direccion del centro de masa, y entre el chasis y esa
      | direccion hay un angulo delta_G. El problema es que delta_G CAMBIA con la postura de las patas: vale 9,09
      | grados con la pata plegada y 1,78 con la pata estirada. O sea que al mover las patas, el cero del angulo
      | se corre mas de 7 grados.
      |
      | Si el firmware no lo compensa, el control cree que el robot esta inclinado cuando no lo esta y sale a
      | corregir: el robot se va 21 cm de donde estaba. Compensando, se queda en cero.
      |
      | Para verlo: poner compensar_delta_G = 0 y mover las patas con un escalon en la consigna de postura.
  estado real : Inport
  postura de las patas : Inport  Port=2
  compensar la postura : Gain  Gain=compensar_delta_G
  delta_G segun la postura : Lookup_n-D  NumberOfTableDimensions=1  BreakpointsForDimension1=tabla_theta  Table=tabla_delta_G  InternalRulePriority=Speed  RndMeth=Simplest
  lo que la IMU informa : Sum  Inputs=+++
  lo que ve el chasis : Sum  Inputs=+-
  phi reconstruido : Sum
  ruido de la IMU : simulink/Sources/Band-Limited White Noise  Cov="[ruido_imu_angulo  ruido_imu_giro]"  Ts=Ts_sensores  seed=[23 29]
  sacar phi y omega de verdad : Gain  Gain=[0 0 1 0; 0 0 0 1]  Multiplication=Matrix(K*u)
  sesgo de la IMU : Constant  Value=[sesgo_imu; 0]
  solo al angulo : Gain  Gain=[1; 0]  Multiplication=Matrix(K*u)
  phi y omega medidos : Outport
  wires:
  estado real/1 -> sacar phi y omega de verdad/1
  postura de las patas/1 -> delta_G segun la postura/1
  delta_G segun la postura/1 -> solo al angulo/1
  sacar phi y omega de verdad/1 -> lo que ve el chasis/1
  solo al angulo/1 -> lo que ve el chasis/2, compensar la postura/1
  lo que ve el chasis/1 -> lo que la IMU informa/1
  ruido de la IMU/1 -> lo que la IMU informa/2
  sesgo de la IMU/1 -> lo que la IMU informa/3
  lo que la IMU informa/1 -> phi reconstruido/1
  compensar la postura/1 -> phi reconstruido/2
  phi reconstruido/1 -> phi y omega medidos/1
